simulink subsystem "MotorDriveUnit_refsub_Basic"  (R2023a)
settings: Solver=VariableStepAuto  StartTime=0.0  StopTime=10.0  RelTol=1e-3
model mask{torque_max=motorDriveUnit.trqMax_Nm, Value=motorDriveUnit.powerMax_kW, Tc=motorDriveUnit.responseTime_s, eff=motorDriveUnit.efficiency_pct, w_eff=motorDriveUnit.spd_eff_rpm, T_eff=motorDriveUnit.trq_eff_Nm, thermal_mass=motorDriveUnit.thermalMass_J_perK, temperature=initial.MDU_Temperature_K, k=motorDriveUnit.dampSpringStiffness_Nm_per_rad, mu_visc=motorDriveUnit.dampSpringFriction_Nm_per_rpm, w_tol=smoothing.MDU_dampSpringVelTol_rpm, T=initial.MDU_AirTemp_K}
  mask prompts: torque_max "Maximum torque [N*m]"; Value "Maximum power [kW]"; Tc "Torque control time constant [s]"; eff "Motor and driver overall efficiency [%]"; w_eff "Speed at which efficiency is measured [rpm]"; T_eff "Torque at which efficiency is measured [N*m]"; thermal_mass "Thermal mass [J/K]"; temperature "Initial temperature [K]"; k "Spring stiffness [N*m/rad]"; mu_visc "Viscous friction coefficient [N*m/rpm]"; w_tol "Velocity tolerance [rpm]"; T "Initial temperature [K]"
undefined symbols (not defined in the file or in its folder): Minus, Plus
libraries: fl_lib x12, nesl_utility x8, sdl_lib x2
settings Model: Creator=isaacito  LastModifiedBy=isaacito
settings SolverCC: AlgebraicLoopSolver=TrustRegion
settings OptimizationCC: ReuseModelBlockBuffer=off
settings DebuggingCC: UnconnectedInputMsg=warning  UnconnectedOutputMsg=warning  UnconnectedLineMsg=warning
settings ModelReferenceCC: EnableRefExpFcnMdlSchedulingChecks=on
settings RTWCC: DLArmComputeVersion=19.05

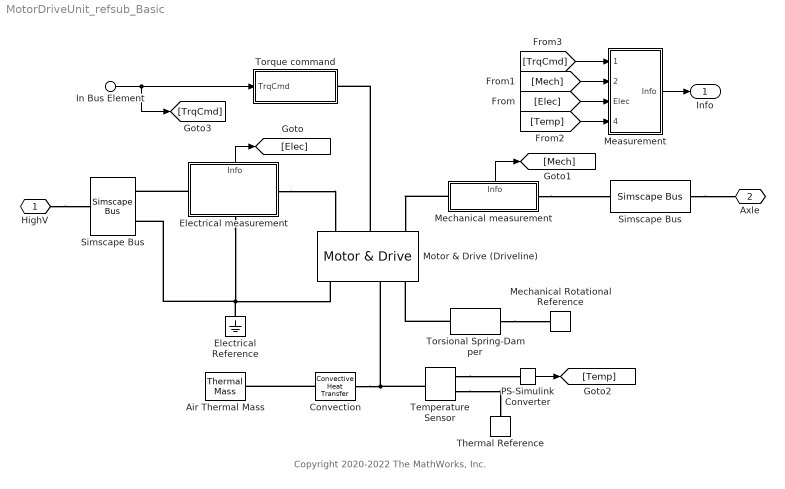
== system MotorDriveUnit_refsub_Basic ==
  note: Copyright 2020-2022 The MathWorks, Inc.
  In Bus Element : Inport  PortName=Ctrl  Element=TrqCmd
      settings: AttributesFormatString=%<Unit>
  " Simscape Bus" : SimscapeBus  HierarchyStrings=Plus;Minus  ConnectionType=Bus: Bus_HighVoltage
  Air Thermal Mass : fl_lib/Thermal/Thermal Elements/Thermal Mass  mass_type=foundation.enum.constant_variable.constant  mass=1000 kg  sp_heat=1000 J/(K*kg)  mass_min=1e-6 kg  num_ports=foundation.enum.numPorts2.one  m_specify=off  m_priority=High  m=1 kg  m_nominal_specify=off  m_nominal_unit=kg  m_nominal_value=1  T_specify=on  T_priority=High  T=T K  T_nominal_specify=off  T_nominal_unit=K  T_nominal_value=1  Q_specify=off  Q_priority=None  Q=0 W  Q_nominal_specify=off  Q_nominal_unit=W  Q_nominal_value=1
      settings: AttributesFormatString=%<T> [%<T_unit>]
  Convection : fl_lib/Thermal/Thermal Elements/Convective Heat Transfer  thermal_type=foundation.enum.constant_variable.constant  area=1 m^2  heat_tr_coeff=20 W/(K*m^2)  min_heat_tr_coeff=1e-3 W/(K*m^2)  T_specify=off  T_priority=None  T=0 K  T_nominal_specify=off  T_nominal_unit=K  T_nominal_value=1  Q_specify=off  Q_priority=None  Q=0 W  Q_nominal_specify=off  Q_nominal_unit=W  Q_nominal_value=1
  Electrical Reference : fl_lib/Electrical/Electrical Elements/Electrical Reference
  Electrical measurement : Subsystem
      settings: PortSchema="{\"entries\":[{\"content\":{\"sides\":[{\"content\":{\"connectorIds\":[\"LConn1\"]},\"type\":\"ConnectorPlacement.EquallySpacedRectSide\",\"uuid\":\"e7899a7c-736a-463f-af66-4f4d60778038\"},{\"content\":{\"connectorIds\":[\"RConn1\"],\"side\":\"RIGHT\"},\"type\":\"ConnectorPlacement.EquallySpacedRectSide\",\"uuid\":\"2a49f66b-d9e4-4ecc-9ee0-ab77c8229b93\"},{\"content\":{\"connectorIds\":[\"Out1\"],\"side\":\"TOP\"},\"type\":\"ConnectorPlacement.EquallySpacedRectSide\",\"uuid\":\"74dc25cc-80bc-4bc6-bed8-e6f8417263f8\"},{\"content\":{\"connectorIds\":[\"RConn2\"],\"side\":\"BOTTOM\"},\"type\":\"ConnectorPlacement.EquallySpacedRectSide\",\"uuid\":\"4e60d196-3559-4d10-956a-034c89d8b166\"}]},\"type\":\"ConnectorPlacement.EquallySpacedConnector\",\"uuid\":\"8c0a083e-e2f2-4f23-9344-a58537a7d46b\"}],\"packageUris\":[\"http://schema.mathworks.com/mf0/Connector/R2020b\"],\"version\":\"1.0\"}"
  Measurement : Subsystem
  Mechanical Rotational Reference : fl_lib/Mechanical/Rotational Elements/Mechanical Rotational Reference
  Mechanical measurement : Subsystem
      settings: PortSchema="{\"entries\":[{\"content\":{\"sides\":[{\"content\":{\"connectorIds\":[\"LConn1\"]},\"type\":\"ConnectorPlacement.EquallySpacedRectSide\",\"uuid\":\"5fa31342-f07e-4673-a9a7-985a7d429b77\"},{\"content\":{\"connectorIds\":[\"RConn1\"],\"side\":\"RIGHT\"},\"type\":\"ConnectorPlacement.EquallySpacedRectSide\",\"uuid\":\"9acd2d80-16ac-46ed-87fd-cbe927805b31\"},{\"content\":{\"connectorIds\":[\"Out1\"],\"side\":\"TOP\"},\"type\":\"ConnectorPlacement.EquallySpacedRectSide\",\"uuid\":\"4cbbe886-3c02-40e0-8c42-e8f0172dc845\"},{\"content\":{\"connectorIds\":[],\"side\":\"HIDDEN\"},\"type\":\"ConnectorPlacement.EquallySpacedRectSide\",\"uuid\":\"587bbe77-2244-497b-b5ee-9581dc02e6d6\"}]},\"type\":\"ConnectorPlacement.EquallySpacedConnector\",\"uuid\":\"7667f692-53dd-486a-a403-194e7923bdd7\"}],\"packageUris\":[\"http://schema.mathworks.com/mf0/Connector/R2020b\"],\"version\":\"1.0\"}"
  Motor & Drive (Driveline) : sdl_lib/Engines & Motors/Motor & Drive  torque_max=torque_max N*m  power_max=Value kW  Tc=Tc s  eff=eff  w_eff=w_eff rpm  T_eff=T_eff N*m  thermal_port=simscape.enum.thermaleffects.model  thermal_mass=thermal_mass J/K  temperature_specify=on  temperature_priority=High  temperature=temperature K  temperature_nominal_specify=off  temperature_nominal_unit=K  temperature_nominal_value=1
      settings: AttributesFormatString=%<temperature> [%<temperature_unit>]  InternalSimscapePortConfiguration="{\"Bottom\":[],\"Left\":[{\"id\":\"Vp\",\"label\":\"+\",\"type\":\"foundation.electrical.electrical\"},{\"id\":\"Tr\",\"label\":\"Tr\",\"type\":\"input\"},{\"id\":\"R\",\"label\":\"R\",\"type\":\"foundation.mechanical.rotational.rotational\"}],\"Right\":[{\"id\":\"Vm\",\"label\":\"-\",\"type\":\"foundation.electrical.electrical\"},{\"id\":\"Omega\",\"label\":\"w\",\"type\":\"output\"},{\"id\":\"H\",\"label\":\"H\",\"type\":\"foundation.thermal.thermal\"},{\"id\":\"C\",\"label\":\"C\",\"type\":\"foundation.mechanical.rotational.rotational\"}],\"Top\":[]}"
  PS-Simulink Converter : nesl_utility/PS-Simulink Converter  PhysicalDomain=network_engine_domain  SubClassName=ps_output  LeftPortType=input  RightPortType=output  PseudoPeriodic=off  Frequencies=[]  VectorFormat=inherit  Unit=K  AffineConversion=on
  Simscape Bus : SimscapeBus  HierarchyStrings=AngSpd  ConnectionType=Bus: Bus_Rotational
  Temperature Sensor : fl_lib/Thermal/Thermal Sensors/Temperature Sensor  temperature_measure=foundation.enum.MeasurementReference.difference
  Thermal Reference : fl_lib/Thermal/Thermal Elements/Thermal Reference
  Torque command : Subsystem
      settings: PortSchema="{\"entries\":[{\"content\":{\"sides\":[{\"content\":{\"connectorIds\":[]},\"type\":\"ConnectorPlacement.EquallySpacedRectSide\",\"uuid\":\"4386e96c-8bc5-4aee-9fb3-c1acfed869a1\"},{\"content\":{\"connectorIds\":[],\"side\":\"RIGHT\"},\"type\":\"ConnectorPlacement.EquallySpacedRectSide\",\"uuid\":\"bdb78bd3-acdc-484f-a422-b6aa6b06314a\"},{\"content\":{\"connectorIds\":[\"In1\"],\"side\":\"TOP\"},\"type\":\"ConnectorPlacement.EquallySpacedRectSide\",\"uuid\":\"e224daec-1fc4-4729-8127-9226b15cc23b\"},{\"content\":{\"connectorIds\":[\"RConn1\"],\"side\":\"BOTTOM\"},\"type\":\"ConnectorPlacement.EquallySpacedRectSide\",\"uuid\":\"92ce3178-8af4-4a3d-bb6e-a8b9ae2a9e27\"}]},\"type\":\"ConnectorPlacement.EquallySpacedConnector\",\"uuid\":\"46cbed77-c00a-44b3-a793-346431068b1b\"}],\"packageUris\":[\"http://schema.mathworks.com/mf0/Connector/R2020b\"],\"version\":\"1.0\"}"
  Torsional Spring-Damper : sdl_lib/Couplings & Drives/Torsional Spring-Damper  k=k N*m/rad  mu_visc=mu_visc m*N/rpm  trq_coulomb=0 N*m  static_kinetic_ratio=1.1  w_tol=w_tol rpm  model_hardstop=0  upper_bound=10 deg  lower_bound=-10 deg  hardstop_model=1  k_endstop=1e6 N*m/rad  D_endstop=10 N*m/(rad/s)  transition=0.001 rad  coeff_rest=0.7  w_tol_hardstop=0.1 rad/s  trq_tol=0.001 N*m  x0=0 deg
      settings: InternalSimscapePortConfiguration="{\"Bottom\":[],\"Left\":[{\"id\":\"R\",\"label\":\"R\",\"type\":\"foundation.mechanical.rotational.rotational\"}],\"Right\":[{\"id\":\"C\",\"label\":\"C\",\"type\":\"foundation.mechanical.rotational.rotational\"}],\"Top\":[]}"
  HighV : PMIOPort  Side=Left
  Axle : PMIOPort  Port=2  Side=Left
  Info : Outport
  wires:
  [TrqCmd] -> Measurement/1(TrqCmd)
  [Temp] -> Measurement/4(Temp)
  Measurement/1(Info) -> Info/1
  [Elec] -> Measurement/3(Elec)
  [Mech] -> Measurement/2(Mech)
  Mechanical measurement/1(Info) -> [Mech]
  Electrical measurement/1(Info) -> [Elec]
  PS-Simulink Converter/1 -> [Temp]
  In Bus Element/1 -> [TrqCmd], Torque command/1(TrqCmd)
  connections:
  " Simscape Bus"/LConn2 -- Motor & Drive (Driveline)/RConn1 -- Electrical measurement/RConn2 -- Electrical Reference/LConn1
  Convection/RConn1 -- Temperature Sensor/LConn1 -- Motor & Drive (Driveline)/RConn3
  Torsional Spring-Damper/RConn1 -- Mechanical Rotational Reference/LConn1
  Torsional Spring-Damper/LConn1 -- Motor & Drive (Driveline)/RConn4
  Motor & Drive (Driveline)/LConn2 -- Torque command/RConn1
  Mechanical measurement/LConn1 -- Motor & Drive (Driveline)/LConn3
  Mechanical measurement/RConn1 -- Simscape Bus/LConn1
  Electrical measurement/RConn1 -- Motor & Drive (Driveline)/LConn1
  Electrical measurement/LConn1 -- " Simscape Bus"/LConn1
  Simscape Bus/RConn1 -- Axle/RConn1
  Convection/LConn1 -- Air Thermal Mass/LConn1
  Temperature Sensor/RConn1 -- Thermal Reference/LConn1
  Temperature Sensor/RConn2 -- PS-Simulink Converter/LConn1
  HighV/RConn1 -- " Simscape Bus"/RConn1

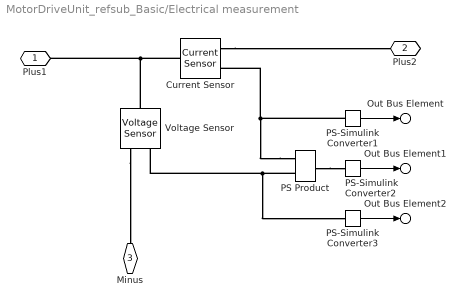
== system MotorDriveUnit_refsub_Basic/Electrical measurement ==
  Current Sensor : fl_lib/Electrical/Electrical Sensors/Current Sensor
  PS Product : fl_lib/Physical Signals/Functions/PS Product
  PS-Simulink Converter1 : nesl_utility/PS-Simulink Converter  PhysicalDomain=network_engine_domain  SubClassName=ps_output  LeftPortType=input  RightPortType=output  PseudoPeriodic=off  Frequencies=[]  VectorFormat=1-D array  Unit=A  AffineConversion=off
  PS-Simulink Converter2 : nesl_utility/PS-Simulink Converter  PhysicalDomain=network_engine_domain  SubClassName=ps_output  LeftPortType=input  RightPortType=output  PseudoPeriodic=off  Frequencies=[]  VectorFormat=1-D array  Unit=kW  AffineConversion=off
  PS-Simulink Converter3 : nesl_utility/PS-Simulink Converter  PhysicalDomain=network_engine_domain  SubClassName=ps_output  LeftPortType=input  RightPortType=output  PseudoPeriodic=off  Frequencies=[]  VectorFormat=1-D array  Unit=V  AffineConversion=off
  Voltage Sensor : fl_lib/Electrical/Electrical Sensors/Voltage Sensor
  Plus1 : PMIOPort  Side=Left
  Plus2 : PMIOPort  Port=2  Side=Right
  Minus : PMIOPort  Port=3  Side=Right
  Out Bus Element : Outport  PortName=Info  Element=Current
  Out Bus Element1 : Outport  PortName=Info  Element=ElecPower
  Out Bus Element2 : Outport  PortName=Info  Element=Voltage
  wires:
  PS-Simulink Converter1/1 -> Out Bus Element/1
  PS-Simulink Converter3/1 -> Out Bus Element2/1
  PS-Simulink Converter2/1 -> Out Bus Element1/1
  connections:
  PS Product/RConn1 -- PS-Simulink Converter2/LConn1
  PS Product/LConn1 -- Current Sensor/RConn1 -- PS-Simulink Converter1/LConn1
  Voltage Sensor/RConn1 -- PS-Simulink Converter3/LConn1 -- PS Product/LConn2
  Voltage Sensor/LConn1 -- Plus1/RConn1 -- Current Sensor/LConn1
  Current Sensor/RConn2 -- Plus2/RConn1
  Voltage Sensor/RConn2 -- Minus/RConn1

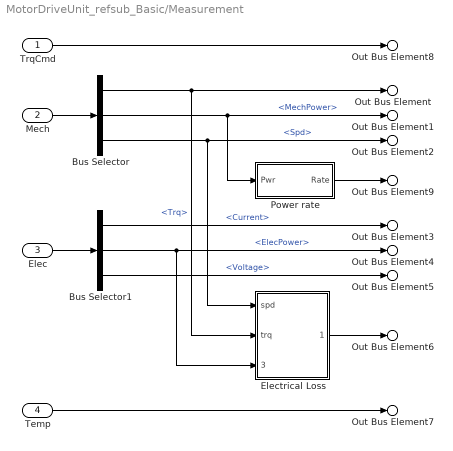
== system MotorDriveUnit_refsub_Basic/Measurement ==
  TrqCmd : Inport
  Mech : Inport  Port=2
  Elec : Inport  Port=3
  Temp : Inport  Port=4
  Bus Selector : BusSelector  OutputSignals=Trq,MechPower,Spd
  Bus Selector1 : BusSelector  OutputSignals=Current,ElecPower,Voltage
  Electrical Loss : Subsystem
  Power rate : Subsystem
  Out Bus Element : Outport  PortName=Info  Element=MotorTrq
  Out Bus Element1 : Outport  PortName=Info  Element=MotorMechPwr
  Out Bus Element2 : Outport  PortName=Info  Element=MotorSpd
  Out Bus Element3 : Outport  PortName=Info  Element=MotorCurrent
  Out Bus Element4 : Outport  PortName=Info  Element=MotorElecPwr
  Out Bus Element5 : Outport  PortName=Info  Element=MotorVoltage
  Out Bus Element6 : Outport  PortName=Info  Element=MotorElecLoss
  Out Bus Element7 : Outport  PortName=Info  Element=MotorTemp
  Out Bus Element8 : Outport  PortName=Info  Element=TrqCmd
  Out Bus Element9 : Outport  PortName=Info  Element=MotorPwrRate
  wires:
  Power rate/1(Rate) -> Out Bus Element9/1
  Temp/1 -> Out Bus Element7/1
  Electrical Loss/1(elec_loss) -> Out Bus Element6/1
  Bus Selector1/3 -> Out Bus Element5/1  "<Voltage>"
  Bus Selector1/2 -> Electrical Loss/3(elec_pwr), Out Bus Element4/1  "<ElecPower>"
  Bus Selector1/1 -> Out Bus Element3/1  "<Current>"
  Bus Selector/3 -> Out Bus Element2/1, Electrical Loss/1(spd)  "<Spd>"
  Bus Selector/2 -> Out Bus Element1/1, Power rate/1(Pwr)  "<MechPower>"
  Bus Selector/1 -> Out Bus Element/1, Electrical Loss/2(trq)  "<Trq>"
  Elec/1 -> Bus Selector1/1
  Mech/1 -> Bus Selector/1
  TrqCmd/1 -> Out Bus Element8/1

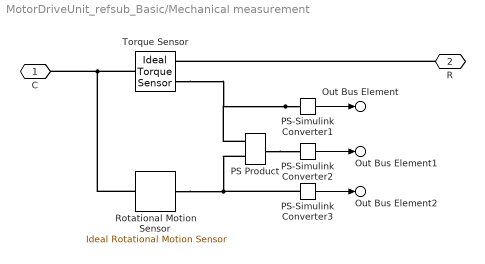
== system MotorDriveUnit_refsub_Basic/Mechanical measurement ==
  PS Product : fl_lib/Physical Signals/Functions/PS Product
  PS-Simulink Converter1 : nesl_utility/PS-Simulink Converter  PhysicalDomain=network_engine_domain  SubClassName=ps_output  LeftPortType=input  RightPortType=output  PseudoPeriodic=off  Frequencies=[]  VectorFormat=1-D array  Unit=N*m  AffineConversion=off
  PS-Simulink Converter2 : nesl_utility/PS-Simulink Converter  PhysicalDomain=network_engine_domain  SubClassName=ps_output  LeftPortType=input  RightPortType=output  PseudoPeriodic=off  Frequencies=[]  VectorFormat=1-D array  Unit=kW  AffineConversion=off
  PS-Simulink Converter3 : nesl_utility/PS-Simulink Converter  PhysicalDomain=network_engine_domain  SubClassName=ps_output  LeftPortType=input  RightPortType=output  PseudoPeriodic=off  Frequencies=[]  VectorFormat=1-D array  Unit=rpm  AffineConversion=off
  Rotational Motion Sensor : fl_lib/Mechanical/Mechanical Sensors/Ideal Rotational Motion Sensor  reference=foundation.enum.MeasurementReference.absolute  acceleration_port=false  velocity_port=true  position_port=false  wrap_angle=simscape.enum.onoff.off  offset=0 rad
      settings: InternalSimscapePortConfiguration="{\"Bottom\":[],\"Left\":[{\"id\":\"R\",\"label\":\"R\",\"type\":\"foundation.mechanical.rotational.rotational\"}],\"Right\":[{\"id\":\"W\",\"label\":\"W\",\"type\":\"output\"}],\"Top\":[]}"
  Torque Sensor : fl_lib/Mechanical/Mechanical Sensors/Ideal Torque Sensor
  C : PMIOPort  Side=Left
  R : PMIOPort  Port=2  Side=Right
  Out Bus Element : Outport  PortName=Info  Element=Trq
  Out Bus Element1 : Outport  PortName=Info  Element=MechPower
  Out Bus Element2 : Outport  PortName=Info  Element=Spd
  wires:
  PS-Simulink Converter1/1 -> Out Bus Element/1
  PS-Simulink Converter2/1 -> Out Bus Element1/1
  PS-Simulink Converter3/1 -> Out Bus Element2/1
  connections:
  PS Product/RConn1 -- PS-Simulink Converter2/LConn1
  PS-Simulink Converter3/LConn1 -- Rotational Motion Sensor/RConn1 -- PS Product/LConn2
  Torque Sensor/LConn1 -- Rotational Motion Sensor/LConn1 -- C/RConn1
  R/RConn1 -- Torque Sensor/RConn1
  PS-Simulink Converter1/LConn1 -- Torque Sensor/RConn2 -- PS Product/LConn1

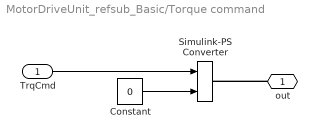
== system MotorDriveUnit_refsub_Basic/Torque command ==
  TrqCmd : Inport
  Constant : Constant  Value=0
  Simulink-PS Converter : nesl_utility/Simulink-PS Converter  PhysicalDomain=network_engine_domain  SubClassName=ps_input  LeftPortType=input  RightPortType=output  PseudoPeriodic=off  Frequencies=[]  NoiseDistribution=none  NoiseParameters=[]  Unit=N*m  AffineConversion=off  FilteringAndDerivatives=provide  SimscapeFilterOrder=1  InputFilterTimeConstant=.001  UdotUserProvided=1
  out : PMIOPort  Side=Right
  wires:
  TrqCmd/1 -> Simulink-PS Converter/1
  Constant/1 -> Simulink-PS Converter/2
  connections:
  out/RConn1 -- Simulink-PS Converter/RConn1

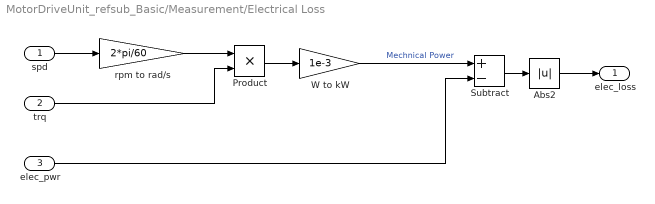
== system MotorDriveUnit_refsub_Basic/Measurement/Electrical Loss ==
  spd : Inport  Unit=rpm
      settings: AttributesFormatString=%<Unit>
  trq : Inport  Port=2  Unit=N*m
      settings: AttributesFormatString=%<Unit>
  elec_pwr : Inport  Port=3  Unit=kW
      settings: AttributesFormatString=%<Unit>
  Abs2 : Abs  ZeroCross=off  SaturateOnIntegerOverflow=off
  Product : Product
  Subtract : Sum  Inputs=+-
  W to kW : Gain  Gain=1e-3
  rpm to rad/s : Gain  Gain=2*pi/60
  elec_loss : Outport  Unit=kW
      settings: AttributesFormatString=%<Unit>
  wires:
  W to kW/1 -> Subtract/1  "Mechnical Power"
  Abs2/1 -> elec_loss/1
  Subtract/1 -> Abs2/1
  elec_pwr/1 -> Subtract/2
  Product/1 -> W to kW/1
  rpm to rad/s/1 -> Product/1
  spd/1 -> rpm to rad/s/1
  trq/1 -> Product/2

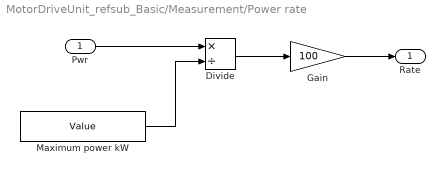
== system MotorDriveUnit_refsub_Basic/Measurement/Power rate ==
  Pwr : Inport  Unit=kW
      settings: AttributesFormatString=%<Unit>
  Divide : Product  Inputs=*/
  Gain : Gain  Gain=100
  Maximum power kW : Constant  Value=Value
  Rate : Outport  Unit=%
  wires:
  Maximum power kW/1 -> Divide/2
  Gain/1 -> Rate/1
  Divide/1 -> Gain/1
  Pwr/1 -> Divide/1
